simulink model "Main"  (R2024a)
settings: Solver=FixedStepAuto  StartTime=0  StopTime=46  FixedStep=0.001  RelTol=1e-3  EnableMultiTasking=on
undefined symbols (not defined in the file): Ab, Ar, C_b, Cdr_off, Cdr_on, Copy_of_AeroTech_O5500X, height_breakpoints2, It, M_b, M_off, M_on, noise_coast, PS, table_data2, velocity_breakpoints2
libraries: simulink x8, aerolibconvert2 x1, simulink_extras x1
settings Model: Creator=simil  LastModifiedBy=simil
settings SolverCC: AutoInsertRateTranBlk=on
settings DataIOCC: FinalStateName=x_at_15_77  InitialState=out.x_at_15_77  SaveOperatingPoint=on  SaveState=on
settings OptimizationCC: DefaultParameterBehavior=Inlined  UseDivisionForNetSlopeComputation=on  GainParamInheritBuiltInType=on  UseFloatMulNetSlope=on  EnhancedBackFolding=on  BooleansAsBitfields=on  PassReuseOutputArgsAs=Individual arguments  StateBitsets=on  DataBitsets=on  ZeroExternalMemoryAtStartup=off  ZeroInternalMemoryAtStartup=off  NoFixptDivByZeroProtection=on  EfficientFloat2IntCast=on  LifeSpan=1  MaxStackSize=64  OptimizeBlockOrder=speed  DifferentSizesBufferReuse=on  EfficientTunableParamExpr=on
settings DebuggingCC: SignalInfNanChecking=error  MultiTaskCondExecSysMsg=none  MultiTaskRateTransMsg=warning  ParamOverflowErrorThreshold=HalfBit  ParameterTunabilityLossMsg=error
settings HardwareCC: ProdBitPerPointer=32  ProdBitPerSizeT=32  ProdBitPerPtrDiffT=32  ProdLargestAtomicInteger=Long  ProdLargestAtomicFloat=Double  ProdWordSize=32  ProdLongLongMode=on  ProdHWDeviceType=ARM Compatible->ARM Cortex-M
settings SFSimCC: MATLABDynamicMemAlloc=off
settings RTWCC: Description=Embedded Coder  SystemTargetFile=ert.tlc  TemplateMakefile=ert_default_tmf  GenerateReport=on  LaunchReport=on  PortableWordSizes=on  GenerateTraceReport=on  GenerateCodeMetricsReport=on
settings CodeAppCC: ForceParamTrailComments=on  IgnoreCustomStorageClasses=off  OperatorAnnotations=on  SimulinkDataObjDesc=on  SFDataObjDesc=on  CustomSymbolStrGlobalVar=rt$N$M  CustomSymbolStrType=$N$M  CustomSymbolStrFcn=$N$M$F  CustomSymbolStrMacro=$N$M  InsertBlockDesc=on
settings ERTTargetCC: TargetLangStandard=C99 (ISO)  CombineSignalStateStructs=on  SupportComplex=off  SupportContinuousTime=on  SupportNonInlinedSFcns=on  ExtModeTransport=3  ExtModeStaticAlloc=on  ExtModeStaticAllocSize=2048  ExtModeMexFile=ext_xcp  ExtModeIntrfLevel=Level2 - Open  RootIOFormat=Structure reference  ERTCustomFileTemplate=example_file_process.tlc  ERTFilePackagingFormat=CompactWithDataFile

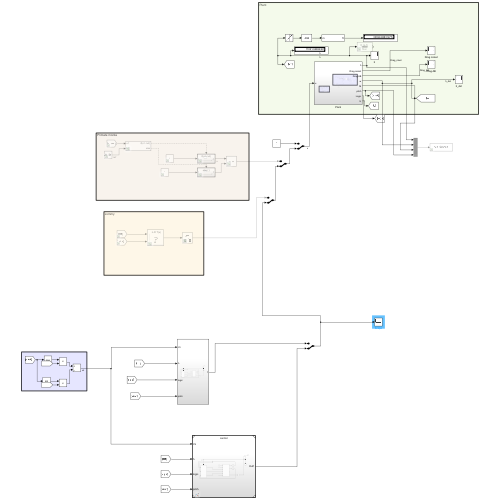
[thumbnail: Simulink's stored preview of the top-level diagram]
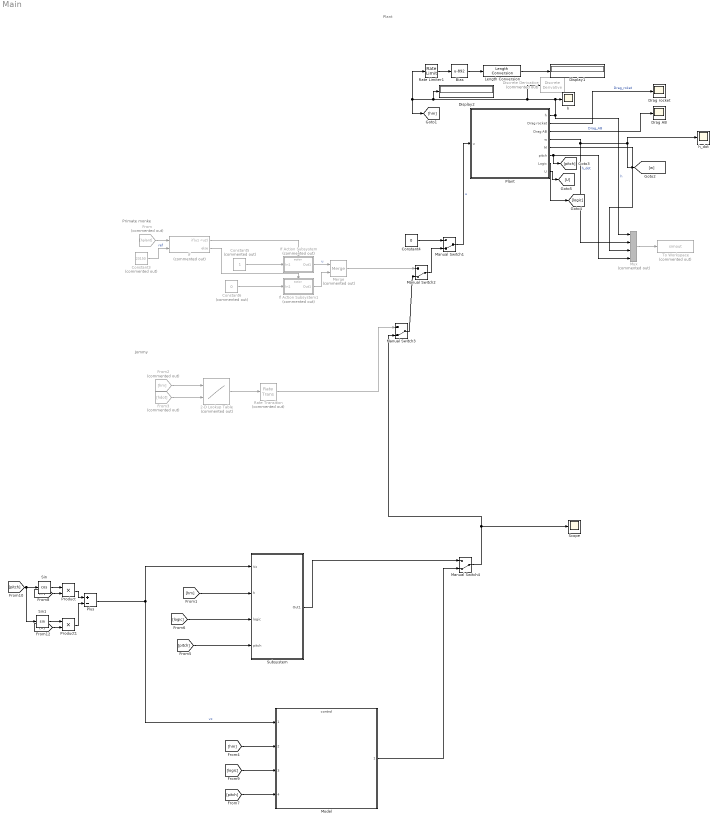
== system Main ==
  note: Jommy
  note: Plant
  note: Primate monke
  2-D Lookup Table : Lookup_n-D  Commented=on  BreakpointsForDimension1=height_breakpoints2  BreakpointsForDimension2=velocity_breakpoints2  Table=table_data2  InterpMethod=Nearest  ExtrapMethod=Clip  RemoveProtectionInput=on  InternalRulePriority=Speed  RndMeth=Simplest
      settings: InputPortMap=u0,u1
  Bias : Bias  Bias=-892  SaturateOnIntegerOverflow=off
  Constant3 : Constant  Commented=on  Value=23150
  Constant4 : Constant  Value=0
  Constant5 : Constant  Commented=on
  Constant6 : Constant  Commented=on  Value=0
  Discrete Derivative : simulink/Discrete/Discrete Derivative  Commented=on  gainval=1.0  ICPrevScaledInput=0.0  OutMin=[]  OutMax=[]  OutDataType=fixdt(1, 16)  OutScaling=2^-10  DoSatur=off
  Display1 : Display
  Display2 : Display
  Drag AB : Scope
  Drag rocket : Scope
  From : From  Commented=on  GotoTag=hplant
  From2 : From  Commented=on  GotoTag=hm
  From3 : From  Commented=on  GotoTag=hdot
  If : If  Commented=on  NumInputs=2  IfExpression=u1 <u2
  If Action Subsystem : Subsystem  Commented=on  TreatAsAtomicUnit=on
  If Action Subsystem1 : Subsystem  Commented=on  TreatAsAtomicUnit=on
  Length Conversion : aerolibconvert2/Length Conversion  IU=m  OU=ft
  Manual Switch{1..4} (4 alike) : ManualSwitch  CurrentSetting=0
  Merge : Merge  Commented=on
  Model : ModelReference  ModelNameDialog=control.slx  SimulationMode=Normal  ModelReferenceVersion=1.2
  Mux : Mux  Commented=on
  Plant : Subsystem
  Plus : Sum  Inputs=+-
  Product : Product
  Product1 : Product
  Rate Limiter1 : RateLimiter  RisingSlewLimit=9999999999999999999999999  FallingSlewLimit=0  SampleTimeMode=inherited
  Rate Transition : RateTransition  Commented=on  OutPortSampleTime=0.05
  Scope : Scope
  Sin : Trigonometry  Operator=cos
  Sin1 : Trigonometry
  Subsystem : Subsystem
  To Workspace : ToWorkspace  Commented=on  VariableName=simout  SaveFormat=Timeseries  SampleTime=0.01
  h : Scope
  h_dot : Scope
  wires:
  Plant/2(Drag rocket) -> Drag rocket/1  "Drag_roket"
  Plant/3(Drag AB) -> Drag AB/1  "Drag_AB"
  Plant/4(w) -> Mux/2, h_dot/1, [w]  "h_dot"
  Rate Limiter1/1 -> Bias/1
  Plant/1(h) -> Discrete Derivative/1, Display2/1, [hm], Rate Limiter1/1, h/1, Mux/1  "h"
  Manual Switch1/1 -> Plant/1(u)  "u"
  From/1 -> If/1
  If Action Subsystem/1(Out1) -> Merge/1  "u"
  Constant4/1 -> Manual Switch1/1
  Constant3/1 -> If/2  "ref"
  If/1 -> If Action Subsystem/Action
  Constant5/1 -> If Action Subsystem/1(In1)
  If/2 -> If Action Subsystem1/Action
  Constant6/1 -> If Action Subsystem1/1(In1)
  If Action Subsystem1/1(Out1) -> Merge/2
  Merge/1 -> Manual Switch2/1
  Manual Switch2/1 -> Manual Switch1/2
  Manual Switch3/1 -> Manual Switch2/2
  2-D Lookup Table/1 -> Rate Transition/1
  From2/1 -> 2-D Lookup Table/1
  From3/1 -> 2-D Lookup Table/2
  Manual Switch4/1 -> Scope/1, Manual Switch3/2
  Rate Transition/1 -> Manual Switch3/1
  Plant/6(pitch) -> [pitch], Mux/4
  Plant/7(Logic) -> [logic]
  Plant/5(M) -> Mux/3
  Mux/1 -> To Workspace/1
  Plant/8(U) -> [U]
  Length Conversion/1 -> Display1/1
  Bias/1 -> Length Conversion/1
  Product1/1 -> Plus/2
  Product/1 -> Plus/1
  [pitch] -> Sin1/1, Sin/1
  [w] -> Product/2
  Sin/1 -> Product/1
  Sin1/1 -> Product1/1
  [U] -> Product1/2
  Plus/1 -> Model/1, Subsystem/1(Vz)  "vz"
  [hm] -> Subsystem/2(h)
  [logic] -> Subsystem/3(logic)
  [pitch] -> Subsystem/4(pitch)
  Subsystem/1(Out1) -> Manual Switch4/1
  Model/1 -> Manual Switch4/2
  [hm] -> Model/2
  [logic] -> Model/3
  [pitch] -> Model/4

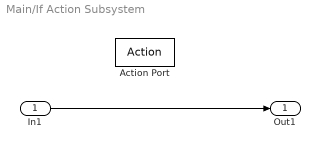
== system Main/If Action Subsystem ==
  In1 : Inport
  Action Port : ActionPort  ActionPortLabel=if(u1 <u2)
  Out1 : Outport
  wires:
  In1/1 -> Out1/1

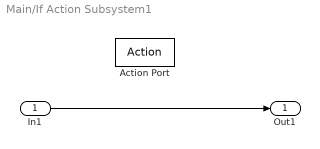
== system Main/If Action Subsystem1 ==
  In1 : Inport
  Action Port : ActionPort  ActionPortLabel=else
  Out1 : Outport
  wires:
  In1/1 -> Out1/1

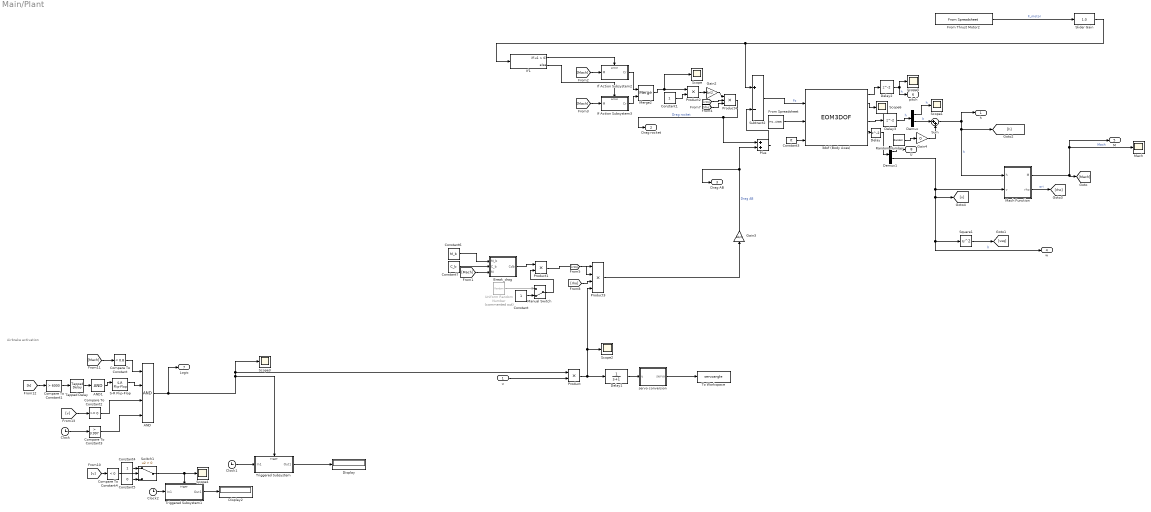
== system Main/Plant ==
  note: Airbrake activation
  u : Inport
  3dof (Body Axes) : EOM3DOF  mtype=Custom Variable  v_ini=0  theta_ini=-6* pi / 180  pos_ini=[0 892]  g=-9.81
  AND : Logic  Inputs=4  IconShape=distinctive  AllPortsSameDT=off  OutDataTypeStr=boolean
  AND1 : Logic  Inputs=1  IconShape=distinctive  AllPortsSameDT=off  OutDataTypeStr=boolean
  Break_drag : MATLAB Function  TreatAsAtomicUnit=on
  Clock : Clock
  Clock1 : Clock
  Clock2 : Clock
  Compare To Constant : simulink/Logic and Bit Operations/Compare To Constant  relop=<  const=0.8  OutDataTypeStr=boolean
  Compare To Constant1 : simulink/Logic and Bit Operations/Compare To Constant  relop=>  const=6000  OutDataTypeStr=boolean
  Compare To Constant2 : simulink/Logic and Bit Operations/Compare To Constant  relop=>=  const=0  OutDataTypeStr=boolean
  Compare To Constant3 : simulink/Logic and Bit Operations/Compare To Constant  relop=>  const=3.997  OutDataTypeStr=boolean
  Compare To Constant4 : simulink/Logic and Bit Operations/Compare To Constant  relop=<  const=0  OutDataTypeStr=boolean
  Constant : Constant
  Constant1 : Constant
  Constant3 : Constant  Value=It
  Constant4 : Constant
  Constant5 : Constant  Value=0
  Constant6 : Constant  Value=M_b
  Constant7 : Constant  Value=C_b
  Delay : Delay
  Delay1 : TransferFcn  Denominator=[1 1]
  Delay2 : Delay
  Delay3 : Delay
  Demux : Demux  Outputs=2
  Demux1 : Demux  Outputs=2
  Display : Display
  Display2 : Display
  From Spreadsheet : FromSpreadsheet  FileName=mass.csv  SheetName=mass  SampleTime=0.001  ExtrapolationBeforeFirstDataPoint=Hold first value  ExtrapolationAfterLastDataPoint=Hold last value
  From Thrust Motor2 : FromSpreadsheet  FileName=Copy_of_AeroTech_O5500X-PS.csv  SheetName=Copy_of_AeroTech_O5500X-PS  OutDataTypeStr=double  SampleTime=0.001  ExtrapolationBeforeFirstDataPoint=Hold first value  ExtrapolationAfterLastDataPoint=Ground value
  Gain2 : Gain  Gain=Ar/2
  Gain3 : Gain  Gain=Ab/2
  Gain4 : Gain  Gain=0
  If Action Subsystem2 : Subsystem  TreatAsAtomicUnit=on
  If Action Subsystem3 : Subsystem  TreatAsAtomicUnit=on
  If1 : If  Priority=2
  Mach : Scope
  Mach Function : MATLAB Function  TreatAsAtomicUnit=on
  Manual Switch : ManualSwitch  CurrentSetting=0
  Merge2 : Merge
  Plus : Sum
  Product : Product
  Product1 : Product
  Product2 : Product
  Product3 : Product  Inputs=4
  Product4 : Product  Inputs=3
  Random Number : RandomNumber  Variance=noise_coast  Seed=randi(538)
  S-R Flip-Flop : simulink_extras/Flip Flops/S-R Flip-Flop  initial_condition=0
  Scope{,1..6} (7 alike) : Scope
  Slider Gain : simulink/Math Operations/Slider Gain  gain=1.0  low=0  high=2
  Square1 : Math  Operator=square
  Subtract2 : Sum  Inputs=+-  RndMeth=Ceiling
  Sum : Sum  Inputs=|++
  Switch1 : Switch  Criteria=u2 > Threshold  SaturateOnIntegerOverflow=off  InputSameDT=off
  Tapped Delay : simulink/Discrete/Tapped Delay  vinit=0  samptime=0.01  NumDelays=3  DelayOrder=Oldest  includeCurrent=on
  To Workspace : ToWorkspace  VariableName=servoangle  SaveFormat=Timeseries  SampleTime=0.3
      settings: Save2DSignal=2-D array (concatenate along first dimension)
  Triggered Subsystem : Subsystem  TreatAsAtomicUnit=on
  Triggered Subsystem1 : Subsystem  TreatAsAtomicUnit=on
  Uniform Random Number : UniformRandomNumber  Commented=on  Minimum=0.7  Maximum=1.5  Seed=rand(1)  SampleTime=0.001
  servo conversion : MATLAB Function  TreatAsAtomicUnit=on
  h : Outport
  Drag rocket : Outport  Port=2
  Drag AB : Outport  Port=3
  w : Outport  Port=4
  M : Outport  Port=5
  pitch : Outport  Port=6
  Logic : Outport  Port=7  OutDataTypeStr=boolean
  U : Outport  Port=8
  wires:
  Product4/1 -> Plus/1, Drag rocket/1  "Drag rocket"
  [rho] -> Product4/3
  From Thrust Motor2/1 -> Slider Gain/1  "F_motor"
  Subtract2/1 -> 3dof (Body Axes)/2  "Fz"
  Square1/1 -> [vsq]
  If1/1 -> If Action Subsystem2/Action
  [vsq] -> Product4/2
  Demux/2 -> Sum/1  "h"
  Gain2/1 -> Product4/1
  Mach Function/1(M) -> M/1, Mach/1, [Mach]  "Mach"
  If Action Subsystem2/1(Cr) -> Merge2/1
  If1/2 -> If Action Subsystem3/Action
  Constant3/1 -> 3dof (Body Axes)/6
  If Action Subsystem3/1(Cr) -> Merge2/2
  [Mach] -> If Action Subsystem2/1(M)
  [Mach] -> If Action Subsystem3/1(M)
  3dof (Body Axes)/4 -> Delay3/1
  Gain3/1 -> Plus/2, Drag AB/1  "Drag AB"
  Mach Function/2(rho) -> [rho]  "ori"
  Plus/1 -> Subtract2/2
  u/1 -> Product/2
  Product3/1 -> Gain3/1
  [vsq] -> Product3/2
  [rho] -> Product3/3
  [Mach] -> Break_drag/3(M)
  Slider Gain/1 -> Subtract2/1, If1/1
  [Mach] -> Compare To Constant/1
  Compare To Constant/1 -> AND/1
  AND1/1 -> S-R Flip-Flop/1
  [v] -> Compare To Constant2/1
  Clock/1 -> Compare To Constant3/1
  Compare To Constant2/1 -> AND/3
  Compare To Constant3/1 -> AND/4
  Clock1/1 -> Triggered Subsystem/1(In1)
  Triggered Subsystem/1(Out1) -> Display/1
  [v] -> Compare To Constant4/1
  Compare To Constant4/1 -> Switch1/2
  Constant4/1 -> Switch1/1
  Constant5/1 -> Switch1/3
  Switch1/1 -> Scope4/1, Triggered Subsystem1/Trigger
  Clock2/1 -> Triggered Subsystem1/1(In1)
  Random Number/1 -> Gain4/1
  3dof (Body Axes)/5 -> Delay/1
  Compare To Constant1/1 -> Tapped Delay/1
  Tapped Delay/1 -> AND1/1
  S-R Flip-Flop/1 -> AND/2
  Gain4/1 -> Sum/2
  Break_drag/1(Cdb) -> Product1/1
  Constant7/1 -> Break_drag/2(C_b)
  Constant6/1 -> Break_drag/1(M_b)
  Product/1 -> Product3/4, Scope2/1, Delay1/1
  AND/1 -> Logic/1, Product/1, Scope3/1, Triggered Subsystem/Trigger
  servo conversion/1(servo) -> To Workspace/1
  Delay1/1 -> servo conversion/1(u)
  3dof (Body Axes)/1 -> Delay2/1
  Delay2/1 -> pitch/1, Scope5/1  "h"
  [h] -> Compare To Constant1/1
  Delay3/1 -> Demux/1  "h"
  Demux/1 -> Scope1/1  "h"
  Delay/1 -> Demux1/1
  Demux1/2 -> w/1, Square1/1, [v], Mach Function/2(v)  "h"
  3dof (Body Axes)/2 -> Scope6/1
  Demux1/1 -> U/1
  Product1/1 -> Product3/1
  Uniform Random Number/1 -> Manual Switch/1
  Merge2/1 -> Scope/1, Product2/1
  Constant1/1 -> Product2/2
  Product2/1 -> Gain2/1
  Constant/1 -> Manual Switch/2
  Manual Switch/1 -> Product1/2
  Sum/1 -> Mach Function/1(h), [h], h/1  "h"
  From Spreadsheet/1 -> 3dof (Body Axes)/4
  Triggered Subsystem1/1(Out1) -> Display2/1

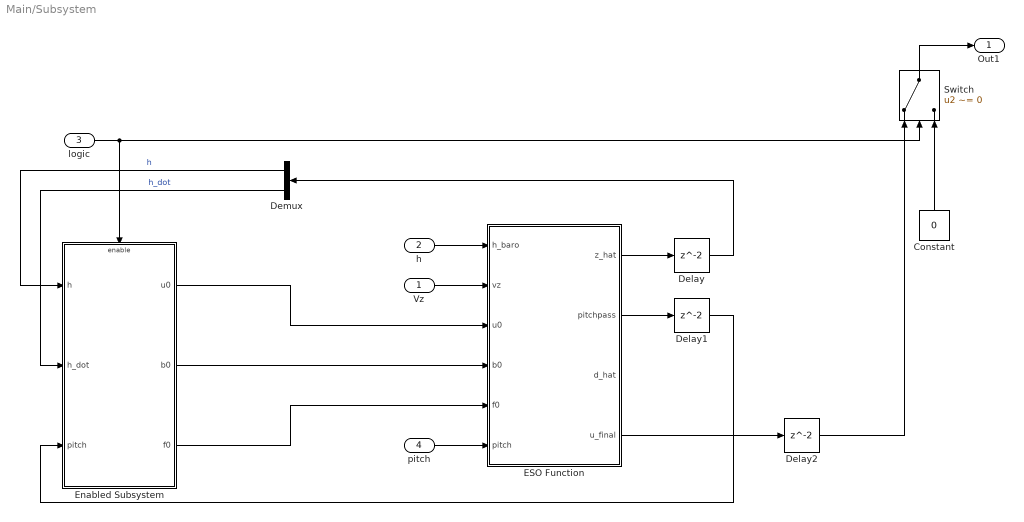
== system Main/Subsystem ==
  Vz : Inport
  h : Inport  Port=2
  logic : Inport  Port=3
  pitch : Inport  Port=4
  Constant : Constant  Value=0
  Delay : Delay
  Delay1 : Delay
  Delay2 : Delay
  Demux : Demux  Outputs=2
  ESO Function : MATLAB Function  TreatAsAtomicUnit=on  SystemSampleTime=0.001
  Enabled Subsystem : Subsystem  TreatAsAtomicUnit=on
  Switch : Switch  Criteria=u2 ~= 0  SaturateOnIntegerOverflow=off  InputSameDT=off
  Out1 : Outport
  wires:
  Vz/1 -> ESO Function/2(vz)
  h/1 -> ESO Function/1(h_baro)
  pitch/1 -> ESO Function/6(pitch)
  logic/1 -> Enabled Subsystem/Enable, Switch/2
  ESO Function/1(z_hat) -> Delay/1
  Delay/1 -> Demux/1
  Demux/1 -> Enabled Subsystem/1(h)  "h"
  Demux/2 -> Enabled Subsystem/2(h_dot)  "h_dot"
  ESO Function/2(pitchpass) -> Delay1/1
  Delay1/1 -> Enabled Subsystem/3(pitch)
  Enabled Subsystem/1(u0) -> ESO Function/3(u0)
  Enabled Subsystem/2(b0) -> ESO Function/4(b0)
  Enabled Subsystem/3(f0) -> ESO Function/5(f0)
  ESO Function/4(u_final) -> Delay2/1
  Constant/1 -> Switch/3
  Delay2/1 -> Switch/1
  Switch/1 -> Out1/1

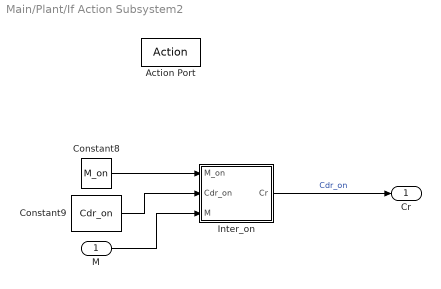
== system Main/Plant/If Action Subsystem2 ==
  M : Inport
  Action Port : ActionPort  ActionPortLabel=if(u1 > 0)
  Constant8 : Constant  Value=M_on
  Constant9 : Constant  Value=Cdr_on
  Inter_on : MATLAB Function  TreatAsAtomicUnit=on
  Cr : Outport
  wires:
  Constant9/1 -> Inter_on/2(Cdr_on)
  Constant8/1 -> Inter_on/1(M_on)
  Inter_on/1(Cr) -> Cr/1  "Cdr_on"
  M/1 -> Inter_on/3(M)

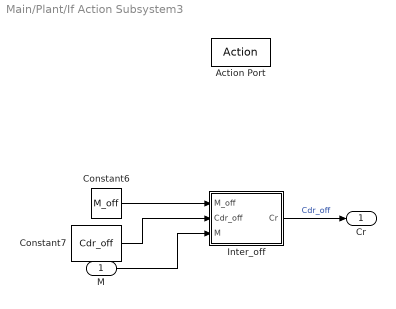
== system Main/Plant/If Action Subsystem3 ==
  M : Inport
  Action Port : ActionPort  ActionPortLabel=else
  Constant6 : Constant  Value=M_off
  Constant7 : Constant  Value=Cdr_off
  Inter_off : MATLAB Function  TreatAsAtomicUnit=on
  Cr : Outport
  wires:
  Constant6/1 -> Inter_off/1(M_off)
  Constant7/1 -> Inter_off/2(Cdr_off)
  M/1 -> Inter_off/3(M)
  Inter_off/1(Cr) -> Cr/1  "Cdr_off"

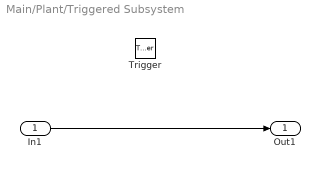
== system Main/Plant/Triggered Subsystem ==
  In1 : Inport
  Trigger : TriggerPort  VariantControl=(inherit)
  Out1 : Outport
  wires:
  In1/1 -> Out1/1

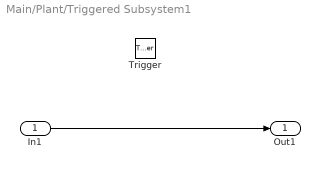
== system Main/Plant/Triggered Subsystem1 ==
  In1 : Inport
  Trigger : TriggerPort  VariantControl=(inherit)
  Out1 : Outport
  wires:
  In1/1 -> Out1/1

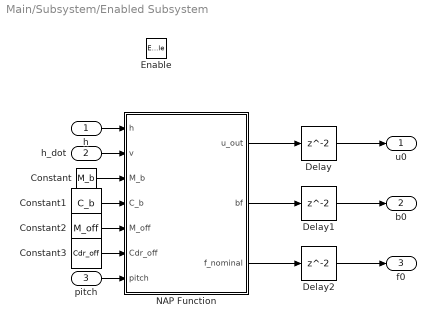
== system Main/Subsystem/Enabled Subsystem ==
  h : Inport
  h_dot : Inport  Port=2
  pitch : Inport  Port=3
  Enable : EnablePort
  Constant : Constant  Value=M_b
  Constant1 : Constant  Value=C_b
  Constant2 : Constant  Value=M_off
  Constant3 : Constant  Value=Cdr_off
  Delay : Delay
  Delay1 : Delay
  Delay2 : Delay
  NAP Function : MATLAB Function  TreatAsAtomicUnit=on  SystemSampleTime=0.01
  u0 : Outport
  b0 : Outport  Port=2
  f0 : Outport  Port=3
  wires:
  Constant/1 -> NAP Function/3(M_b)
  Constant2/1 -> NAP Function/5(M_off)
  Constant3/1 -> NAP Function/6(Cdr_off)
  Constant1/1 -> NAP Function/4(C_b)
  h/1 -> NAP Function/1(h)
  h_dot/1 -> NAP Function/2(v)
  pitch/1 -> NAP Function/7(pitch)
  NAP Function/1(u_out) -> Delay/1
  NAP Function/2(bf) -> Delay1/1
  NAP Function/3(f_nominal) -> Delay2/1
  Delay/1 -> u0/1
  Delay1/1 -> b0/1
  Delay2/1 -> f0/1

== matlab function Main/Plant/If Action Subsystem2/Inter_on ==
  data: M_on input; Cdr_on input; M input; Cr output
function Cr = fcn(M_on,Cdr_on,M)
Cr = interp1(M_on,Cdr_on,M,"linear", 'extrap');
Cr(isnan(Cr)) = 0.3783986725;
end

== matlab function Main/Plant/Mach Function ==
  data: h input; v input; M output; rho output
function [M,rho] = Mach(h,v)

if isnan(h) || isnan(v)
    M = 0; rho = 1.225; 
    return;
end
% --- ISA Constants (Precision alignment) ---
L = 0.0065;       % Temperature lapse rate [K/m]
T0 = 288.15;      % Sea level temperature [K]
P0 = 101325;      % Sea level pressure [Pa]
R = 287.0528;     % Gas constant for air [J/kg*K]
gamma = 1.4;      % Ratio of specific heats

% --- Physics Calculations ---
T = T0 - L * h;                               % Temperature at altitude
c = sqrt(gamma * R * T);                      % Speed of sound
M = v / c;                                % Mach number
P = P0 * (T / T0)^5.2558; 
rho = P / (R * T);                            

end

== matlab function Main/Plant/If Action Subsystem3/Inter_off ==
  data: M_off input; Cdr_off input; M input; Cr output
function Cr = fcn(M_off,Cdr_off,M)

Cr = interp1(M_off,Cdr_off,M,"linear", 'extrap');
Cr(isnan(Cr)) = 0.3783986725;
% Cr(iszero(Cr)) = 
end

== matlab function Main/Plant/servo conversion ==
  data: u input; servo output
function servo = fcn(u)
servo_i = 160.5;
servo_f = 24.5;
servo =  (servo_f-servo_i)*u + servo_i;
end

== matlab function Main/Plant/Break_drag ==
  data: M_b input; C_b input; M input; Cdb output
function Cdb = fcn(M_b,C_b,M)
%#codegen
Cdb = interp1(M_b,C_b,M,"linear", 'extrap');
Cdb(isnan(Cdb)) = 0;
end

== matlab function Main/Subsystem/ESO Function ==
  data: h_baro input; z_hat output; pitchpass output; vz input; u0 input; b0 input; f0 input; pitch input; d_hat output; u_final output
function [z_hat,pitchpass,d_hat, u_final] = fcn(h_baro, vz, u0, b0, f0, pitch)
%#codegen
omega = 6;
if isnan(u0), u0 = 0; end
if isnan(b0) || b0 == 0, b0 = -5; end
if isnan(f0), f0 = -9.81; end
pitchpass = pitch;

persistent z1 z2 z3 u_prev
stepsize = 0.001;
if isempty(z1)
    z1 = 892; z2 = 0; z3 = -9.81; u_prev = 0;
    if ~isnan(h_baro), z1 = h_baro; end
    if ~isnan(vz), z2 = vz; end
    if ~isnan(f0), z3 = f0; end
end

if isnan(h_baro) || isnan(vz)
    z_hat = [z1; z2];
    d_hat = z3;
    u_final = u_prev;
else
    beta1 = 3 * omega;
    beta2 = 3 * (omega^2);
    beta3 = omega^3;
    e = z1 - h_baro;
    max_rate = 0.3;
    delta_correction = max(-0.5, min(0.5, -z3 / b0));
    u_raw = u0 + delta_correction;
    u_ratelimited = u_prev + max(min(u_raw - u_prev, max_rate), -max_rate);
    u_final = max(0.0, min(1.0, u_ratelimited));

    z1_next = z1 + stepsize*(z2 - beta1*e);
    z2_next = z2 + stepsize*(z3 + f0 - beta2*e + b0*u_final);
    z3_next = z3 + stepsize*(-beta3*e);
    z1 = z1_next;
    z2 = z2_next;
    z3 = z3_next;
    u_prev = u_final;
    z_hat = [z1; z2];
    d_hat = z3;
end
end

== matlab function Main/Subsystem/Enabled Subsystem/NAP Function ==
  settings: updateMethod=DISCRETE
  data: h input; u_out output; v input; M_b input; C_b input; M_off input; Cdr_off input; pitch input; bf output; f_nominal output
function [u_out,bf,f_nominal] = NAP(h,v,M_b,C_b,M_off,Cdr_off,pitch)
    u_out = 0; 
    bf = -4.5;
    f_nominal = -9.81;
    persistent tick u_store bf_store f_store

    if isempty(tick)
        tick = 0;    
        u_store = 0;
        bf_store = bf;
        f_store = f_nominal;
    end

    if isnan(h) || isnan(v)
       return
    end

if tick <= 0
    h_target = (33400)*0.3048+892;
    [h_pred_min,bf_min,f_min] = RK2(h, v, pitch, 0.0, M_b, C_b, M_off, Cdr_off);
    
    if h_pred_min < h_target
        u_out = 0.0;
        bf = bf_min;
        f_nominal = f_min;
        return;
    end
    [h_pred_max,bf_max,f_max] = RK2(h, v, pitch, 1.0, M_b, C_b, M_off, Cdr_off);
    if h_pred_max > h_target
        u_out = 1.0;
        bf = bf_max;
        f_nominal = f_max;
        return;
    end

    u_low = 0.0;
    u_high = 1.0;
    u_mid = 0.5;

    for iter = 1:5
        [h_sim,current_bf,current_f] = RK2(h, v, pitch, u_mid, M_b, C_b, M_off, Cdr_off);
        bf_store = current_bf;
        f_store = current_f;
        if h_sim > h_target
            u_low = u_mid;
        else
            u_high = u_mid;
        end
        u_mid = (u_low + u_high) / 2;
    end
    u_out = u_mid; 
    u_store = u_out;
    tick = 10;
end
    tick = tick - 1;
    u_out = u_store;
    bf = bf_store;
    f_nominal = f_store;
end

function [h_final,bf,f] = RK2(h, v, pitch, u_val, M_b, C_b, M_off, Cdr_off)
    m = 25.142; Ar = pi*(0.131/2)^2; Ab = 2*1111.162e-6; g = 9.81;         
    dt = 0.1;      
    h1 = h;
    v1 = v;
    stream0 = v / cos(pitch);
    T0 = 288.15 - 0.0065 * h;
    P0 = 101325 * (T0 / 288.15)^5.2558;
    rho0 = P0 / (287.0528 * T0);
    mach0 = stream0/sqrt(1.4*287.0528*T0);
    Cdb0 = interp1(M_b, C_b, mach0, 'linear', 'extrap');
    Cdr0 = interp1(M_off, Cdr_off, mach0, 'linear', 'extrap');
    bf = (-0.5 * rho0 * stream0^2 * Cdb0 * Ab / m) * cos(pitch);
    f = (-0.5 * rho0 * stream0^2 * Cdr0 * Ar / m) * cos(pitch) - g;
   
    max_iter = 500;
    for iter_rk = 1:max_iter
        if v1 < 0, break; end
        stream1 = v1/cos(pitch);
        T1 = 288.15 - 0.0065 * h1;
        P1 = 101325 * (T1 / 288.15)^5.2558;
        rho1 = P1 / (287.0528 * T1);
        mach1 = stream1 / sqrt(1.4 * 287.0528 * T1);
        Cdb1 = interp1(M_b, C_b, mach1, 'linear', 'extrap');
        Cdr1 = interp1(M_off, Cdr_off, mach1, 'linear', 'extrap');
        b0_1 = (-0.5 * rho1 * stream1^2 * Cdb1 * Ab / m) * cos(pitch);
        f1 = (-0.5 * rho1 * stream1^2 * Cdr1 * Ar / m) * cos(pitch) - g;
        a1 = f1 + b0_1 * u_val; 
        h2 = h1 + v1 * (dt / 2);
        v2 = v1 + a1 * (dt / 2);
        stream2 = v2/cos(pitch);
        T2 = 288.15 - 0.0065 * h2;
        P2 = 101325 * (T2 / 288.15)^5.2558;
        rho2 = P2 / (287.0528 * T2);
        mach2 = stream2 / sqrt(1.4 * 287.0528 * T2);
        Cdb2 = interp1(M_b, C_b, mach2, 'linear', 'extrap');
        Cdr2 = interp1(M_off, Cdr_off, mach2, 'linear', 'extrap');
        b0_2 = (-0.5 * rho2 * stream2^2 * Cdb2 * Ab / m) * cos(pitch);
        f2 = (-0.5 * rho2 * stream2^2 * Cdr2 * Ar / m) * cos(pitch) - g;
        a2 = f2 + b0_2 * u_val; 
        v1 = v1 + a2 * dt;
        h1 = h1 + v2 * dt;
        if h1 > 12000, break; end
    end
    h_final = h1;
end
